simulink library "three_phase_bridge_three_level_ttype_ideal_switch"  (R2026a)
settings: Solver=VariableStepAuto
libraries: fl_lib x60, nesl_utility x36
settings Model: Creator=pwr-control  LastModifiedBy=pwr-control

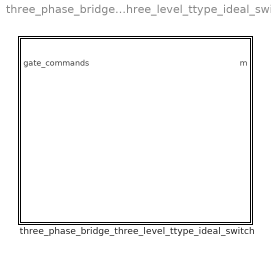
== system three_phase_bridge_three_level_ttype_ideal_switch ==
  three_phase_bridge_three_level_ttype_ideal_switch : Subsystem  mask(three_phase_bridge_three_level_ttype_ideal_switch){Rds_on=1.85e-3, Vdon_diode=0.35, Rdon_diode=1.85e-3, Csnubber=6e-9, Rsnubber=3e3, Vth=7.5}
      mask prompts: Rds_on "On-state resistance of the switch [Ohm]"; Vdon_diode "Diode forward voltage [V]"; Rdon_diode "Diode on-state resistance [Ohm]"; Csnubber "RC snubber capacitance [F]"; Rsnubber "RC snubber resistance [Ohm]"; Vth "Gate threshold: the switch is closed when the gate command is above Vth"
      mask help: Three-phase bridge, three-level T-type, ideal switch devices. Ideal switch cells: Simscape Foundation controlled switch (closed when the gate command is above Vth) with antiparallel piecewise-linear diode and RC snubber. No losses are computed; the cell measures the device current (positive from collector/drain to emitter/source, diode current negative) and the device voltage. Bus m: switch_current_Qk, switch_voltage_Qk. Ports: gate_commands (bus from the three-level PWM modulators of masked_models/modulators), m (measurement bus), left dc terminals udc(+) / np / udc(-), right ac terminals u / v / w. Device numbering: see three_phase_bridge/README.md.
      mask Help: web('https://github.com/pwr-control/library/blob/dev/library/masked_models/semiconductors_bridges/three_phase_bridge/README.md', '-browser')
      mask DialogControl ParameterGroupVar Prompt: Switch and diode
      mask DialogControl ParameterGroupVar1 Prompt: RC snubber
      mask Display:
      | disp(sprintf('three-phase bridge\nT-type 3 levels\nideal switch'))
      | port_label('input', 1, 'gate_commands')
      | port_label('output', 1, 'm')
      | port_label('LConn', 1, 'udc(+)')
      | port_label('LConn', 2, 'np')
      | port_label('LConn', 3, 'udc(-)')
      | port_label('RConn', 1, 'u')
      | port_label('RConn', 2, 'v')
      | port_label('RConn', 3, 'w')

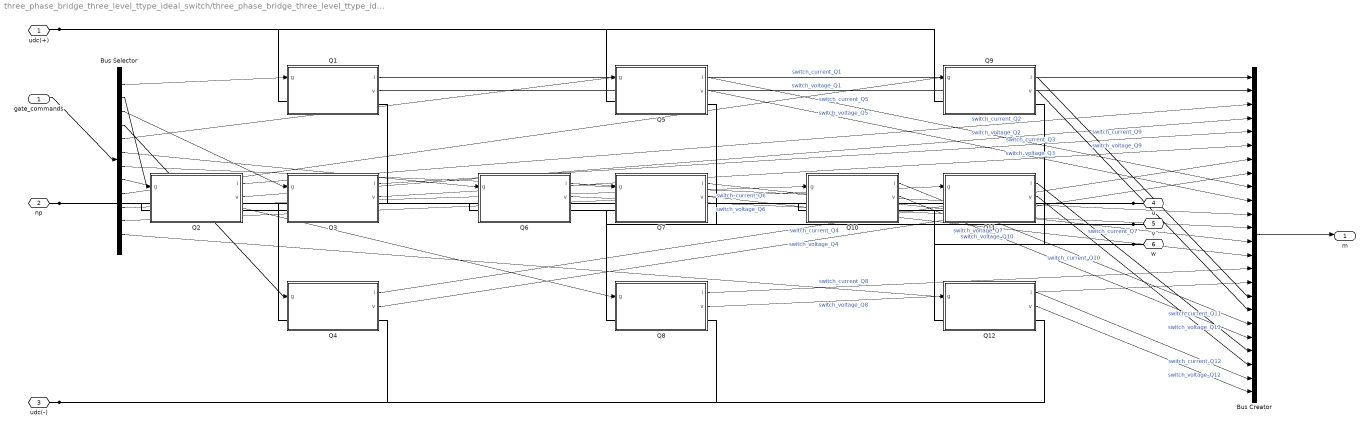
== system three_phase_bridge_three_level_ttype_ideal_switch/three_phase_bridge_three_level_ttype_ideal_switch ==
  gate_commands : Inport
  Bus Selector : BusSelector  OutputSignals=gate_cmds_phu.cmd_gate_Q1,gate_cmds_phu.cmd_gate_Q2,gate_cmds_phu.cmd_gate_Q3,gate_cmds_phu.cmd_gate_Q4,gate_cmds_phv.cmd_gate_Q1,gate_cmds_phv.cmd_gate_Q2,gate_cmds_phv.cmd_gate_Q3,gate_cmds_phv.cmd_gate_Q4,gate_cmds_phw.cmd_gate_Q1,gate_cmds_phw.cmd_gate_Q2,gate_cmds_phw.cmd_gate_Q3,gate_cmds_phw.cmd_gate_Q4
  udc(+) : PMIOPort  Side=Left
  np : PMIOPort  Port=2  Side=Left
  udc(-) : PMIOPort  Port=3  Side=Left
  u : PMIOPort  Port=4  Side=Right
  v : PMIOPort  Port=5  Side=Right
  w : PMIOPort  Port=6  Side=Right
  Bus Creator : BusCreator  Inputs=24
  m : Outport
  Q1 : Subsystem
  Q2 : Subsystem
  Q3 : Subsystem
  Q4 : Subsystem
  Q5 : Subsystem
  Q6 : Subsystem
  Q7 : Subsystem
  Q8 : Subsystem
  Q9 : Subsystem
  Q10 : Subsystem
  Q11 : Subsystem
  Q12 : Subsystem
  wires:
  gate_commands/1 -> Bus Selector/1
  Bus Creator/1 -> m/1
  Bus Selector/1 -> Q1/1(g)
  Q1/1(i) -> Bus Creator/1  "switch_current_Q1"
  Q1/2(v) -> Bus Creator/2  "switch_voltage_Q1"
  Bus Selector/2 -> Q2/1(g)
  Q2/1(i) -> Bus Creator/3  "switch_current_Q2"
  Q2/2(v) -> Bus Creator/4  "switch_voltage_Q2"
  Bus Selector/3 -> Q3/1(g)
  Q3/1(i) -> Bus Creator/5  "switch_current_Q3"
  Q3/2(v) -> Bus Creator/6  "switch_voltage_Q3"
  Bus Selector/4 -> Q4/1(g)
  Q4/1(i) -> Bus Creator/7  "switch_current_Q4"
  Q4/2(v) -> Bus Creator/8  "switch_voltage_Q4"
  Bus Selector/5 -> Q5/1(g)
  Q5/1(i) -> Bus Creator/9  "switch_current_Q5"
  Q5/2(v) -> Bus Creator/10  "switch_voltage_Q5"
  Bus Selector/6 -> Q6/1(g)
  Q6/1(i) -> Bus Creator/11  "switch_current_Q6"
  Q6/2(v) -> Bus Creator/12  "switch_voltage_Q6"
  Bus Selector/7 -> Q7/1(g)
  Q7/1(i) -> Bus Creator/13  "switch_current_Q7"
  Q7/2(v) -> Bus Creator/14  "switch_voltage_Q7"
  Bus Selector/8 -> Q8/1(g)
  Q8/1(i) -> Bus Creator/15  "switch_current_Q8"
  Q8/2(v) -> Bus Creator/16  "switch_voltage_Q8"
  Bus Selector/9 -> Q9/1(g)
  Q9/1(i) -> Bus Creator/17  "switch_current_Q9"
  Q9/2(v) -> Bus Creator/18  "switch_voltage_Q9"
  Bus Selector/10 -> Q10/1(g)
  Q10/1(i) -> Bus Creator/19  "switch_current_Q10"
  Q10/2(v) -> Bus Creator/20  "switch_voltage_Q10"
  Bus Selector/11 -> Q11/1(g)
  Q11/1(i) -> Bus Creator/21  "switch_current_Q11"
  Q11/2(v) -> Bus Creator/22  "switch_voltage_Q11"
  Bus Selector/12 -> Q12/1(g)
  Q12/1(i) -> Bus Creator/23  "switch_current_Q12"
  Q12/2(v) -> Bus Creator/24  "switch_voltage_Q12"
  connections:
  Q2/RConn1 -- Q3/RConn1
  u/RConn1 -- Q1/RConn1 -- Q4/LConn1 -- Q3/LConn1
  Q6/RConn1 -- Q7/RConn1
  v/RConn1 -- Q5/RConn1 -- Q8/LConn1 -- Q7/LConn1
  Q10/RConn1 -- Q11/RConn1
  w/RConn1 -- Q9/RConn1 -- Q12/LConn1 -- Q11/LConn1
  udc(+)/RConn1 -- Q1/LConn1 -- Q5/LConn1 -- Q9/LConn1
  udc(-)/RConn1 -- Q4/RConn1 -- Q8/RConn1 -- Q12/RConn1
  np/RConn1 -- Q2/LConn1 -- Q6/LConn1 -- Q10/LConn1

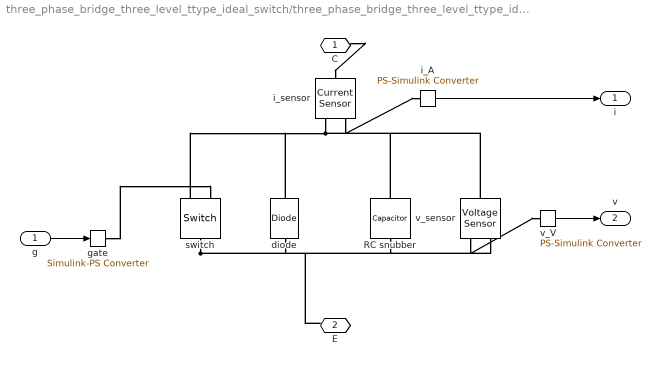
== system three_phase_bridge_three_level_ttype_ideal_switch/three_phase_bridge_three_level_ttype_ideal_switch/Q1 ==
  g : Inport
  gate : nesl_utility/Simulink-PS Converter  PhysicalDomain=network_engine_domain  SubClassName=ps_input  LeftPortType=input  RightPortType=output  PseudoPeriodic=off  Frequencies=[]  NoiseDistribution=none  NoiseParameters=[]  Unit=1  AffineConversion=off  FilteringAndDerivatives=provide  SimscapeFilterOrder=1  InputFilterTimeConstant=0.001  UdotUserProvided=0
  C : PMIOPort  Side=Left
  i_sensor : fl_lib/Electrical/Electrical Sensors/Current Sensor
  switch : fl_lib/Electrical/Electrical Elements/Switch  R_closed=Rds_on Ohm  G_open=1e-8 1/Ohm  Threshold=Vth  i_specify=off  i_priority=None  i=0 A  i_nominal_specify=off  i_nominal_value=1  i_nominal_unit=A  v_specify=off  v_priority=None  v=0 V  v_nominal_specify=off  v_nominal_value=1  v_nominal_unit=V
  diode : fl_lib/Electrical/Electrical Elements/Diode  Vf=Vdon_diode V  Ron=Rdon_diode Ohm  Goff=1e-8 1/Ohm  i_specify=off  i_priority=None  i=0 A  i_nominal_specify=off  i_nominal_value=1  i_nominal_unit=A  v_specify=off  v_priority=None  v=0 V  v_nominal_specify=off  v_nominal_value=1  v_nominal_unit=V
  RC snubber : fl_lib/Electrical/Electrical Elements/Capacitor  c=Csnubber F  r=Rsnubber Ohm  g=0 1/Ohm  i_specify=off  i_priority=None  i=0 A  i_nominal_specify=off  i_nominal_value=1  i_nominal_unit=A  v_specify=off  v_priority=None  v=0 V  v_nominal_specify=off  v_nominal_value=1  v_nominal_unit=V  vc_specify=off  vc_priority=High  vc=0 V  vc_nominal_specify=off  vc_nominal_value=1  vc_nominal_unit=V
  v_sensor : fl_lib/Electrical/Electrical Sensors/Voltage Sensor
  E : PMIOPort  Port=2  Side=Right
  i_A : nesl_utility/PS-Simulink Converter  PhysicalDomain=network_engine_domain  SubClassName=ps_output  LeftPortType=input  RightPortType=output  PseudoPeriodic=off  Frequencies=[]  VectorFormat=1-D array  Unit=A  AffineConversion=off
  v_V : nesl_utility/PS-Simulink Converter  PhysicalDomain=network_engine_domain  SubClassName=ps_output  LeftPortType=input  RightPortType=output  PseudoPeriodic=off  Frequencies=[]  VectorFormat=1-D array  Unit=V  AffineConversion=off
  i : Outport
  v : Outport  Port=2
  wires:
  g/1 -> gate/1
  i_A/1 -> i/1
  v_V/1 -> v/1
  connections:
  gate/RConn1 -- switch/RConn1
  C/RConn1 -- i_sensor/LConn1
  i_sensor/RConn2 -- switch/RConn2 -- diode/RConn1 -- RC snubber/LConn1 -- v_sensor/LConn1
  switch/LConn1 -- diode/LConn1 -- RC snubber/RConn1 -- v_sensor/RConn2 -- E/RConn1
  i_sensor/RConn1 -- i_A/LConn1
  v_sensor/RConn1 -- v_V/LConn1

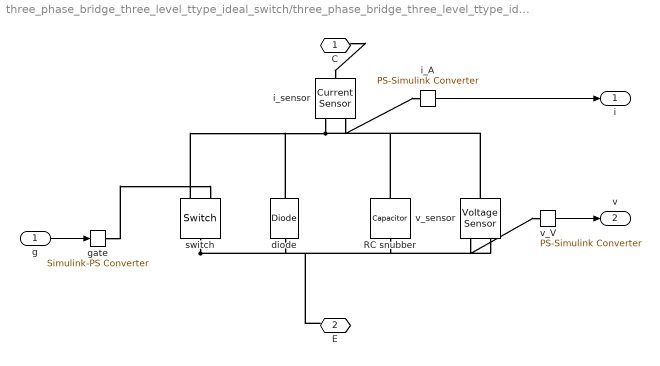
== system three_phase_bridge_three_level_ttype_ideal_switch/three_phase_bridge_three_level_ttype_ideal_switch/Q2 ==
  g : Inport
  gate : nesl_utility/Simulink-PS Converter  PhysicalDomain=network_engine_domain  SubClassName=ps_input  LeftPortType=input  RightPortType=output  PseudoPeriodic=off  Frequencies=[]  NoiseDistribution=none  NoiseParameters=[]  Unit=1  AffineConversion=off  FilteringAndDerivatives=provide  SimscapeFilterOrder=1  InputFilterTimeConstant=0.001  UdotUserProvided=0
  C : PMIOPort  Side=Left
  i_sensor : fl_lib/Electrical/Electrical Sensors/Current Sensor
  switch : fl_lib/Electrical/Electrical Elements/Switch  R_closed=Rds_on Ohm  G_open=1e-8 1/Ohm  Threshold=Vth  i_specify=off  i_priority=None  i=0 A  i_nominal_specify=off  i_nominal_value=1  i_nominal_unit=A  v_specify=off  v_priority=None  v=0 V  v_nominal_specify=off  v_nominal_value=1  v_nominal_unit=V
  diode : fl_lib/Electrical/Electrical Elements/Diode  Vf=Vdon_diode V  Ron=Rdon_diode Ohm  Goff=1e-8 1/Ohm  i_specify=off  i_priority=None  i=0 A  i_nominal_specify=off  i_nominal_value=1  i_nominal_unit=A  v_specify=off  v_priority=None  v=0 V  v_nominal_specify=off  v_nominal_value=1  v_nominal_unit=V
  RC snubber : fl_lib/Electrical/Electrical Elements/Capacitor  c=Csnubber F  r=Rsnubber Ohm  g=0 1/Ohm  i_specify=off  i_priority=None  i=0 A  i_nominal_specify=off  i_nominal_value=1  i_nominal_unit=A  v_specify=off  v_priority=None  v=0 V  v_nominal_specify=off  v_nominal_value=1  v_nominal_unit=V  vc_specify=off  vc_priority=High  vc=0 V  vc_nominal_specify=off  vc_nominal_value=1  vc_nominal_unit=V
  v_sensor : fl_lib/Electrical/Electrical Sensors/Voltage Sensor
  E : PMIOPort  Port=2  Side=Right
  i_A : nesl_utility/PS-Simulink Converter  PhysicalDomain=network_engine_domain  SubClassName=ps_output  LeftPortType=input  RightPortType=output  PseudoPeriodic=off  Frequencies=[]  VectorFormat=1-D array  Unit=A  AffineConversion=off
  v_V : nesl_utility/PS-Simulink Converter  PhysicalDomain=network_engine_domain  SubClassName=ps_output  LeftPortType=input  RightPortType=output  PseudoPeriodic=off  Frequencies=[]  VectorFormat=1-D array  Unit=V  AffineConversion=off
  i : Outport
  v : Outport  Port=2
  wires:
  g/1 -> gate/1
  i_A/1 -> i/1
  v_V/1 -> v/1
  connections:
  gate/RConn1 -- switch/RConn1
  C/RConn1 -- i_sensor/LConn1
  i_sensor/RConn2 -- switch/RConn2 -- diode/RConn1 -- RC snubber/LConn1 -- v_sensor/LConn1
  switch/LConn1 -- diode/LConn1 -- RC snubber/RConn1 -- v_sensor/RConn2 -- E/RConn1
  i_sensor/RConn1 -- i_A/LConn1
  v_sensor/RConn1 -- v_V/LConn1

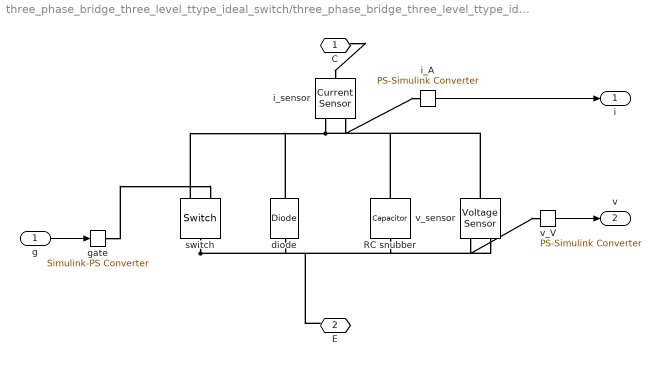
== system three_phase_bridge_three_level_ttype_ideal_switch/three_phase_bridge_three_level_ttype_ideal_switch/Q3 ==
  g : Inport
  gate : nesl_utility/Simulink-PS Converter  PhysicalDomain=network_engine_domain  SubClassName=ps_input  LeftPortType=input  RightPortType=output  PseudoPeriodic=off  Frequencies=[]  NoiseDistribution=none  NoiseParameters=[]  Unit=1  AffineConversion=off  FilteringAndDerivatives=provide  SimscapeFilterOrder=1  InputFilterTimeConstant=0.001  UdotUserProvided=0
  C : PMIOPort  Side=Left
  i_sensor : fl_lib/Electrical/Electrical Sensors/Current Sensor
  switch : fl_lib/Electrical/Electrical Elements/Switch  R_closed=Rds_on Ohm  G_open=1e-8 1/Ohm  Threshold=Vth  i_specify=off  i_priority=None  i=0 A  i_nominal_specify=off  i_nominal_value=1  i_nominal_unit=A  v_specify=off  v_priority=None  v=0 V  v_nominal_specify=off  v_nominal_value=1  v_nominal_unit=V
  diode : fl_lib/Electrical/Electrical Elements/Diode  Vf=Vdon_diode V  Ron=Rdon_diode Ohm  Goff=1e-8 1/Ohm  i_specify=off  i_priority=None  i=0 A  i_nominal_specify=off  i_nominal_value=1  i_nominal_unit=A  v_specify=off  v_priority=None  v=0 V  v_nominal_specify=off  v_nominal_value=1  v_nominal_unit=V
  RC snubber : fl_lib/Electrical/Electrical Elements/Capacitor  c=Csnubber F  r=Rsnubber Ohm  g=0 1/Ohm  i_specify=off  i_priority=None  i=0 A  i_nominal_specify=off  i_nominal_value=1  i_nominal_unit=A  v_specify=off  v_priority=None  v=0 V  v_nominal_specify=off  v_nominal_value=1  v_nominal_unit=V  vc_specify=off  vc_priority=High  vc=0 V  vc_nominal_specify=off  vc_nominal_value=1  vc_nominal_unit=V
  v_sensor : fl_lib/Electrical/Electrical Sensors/Voltage Sensor
  E : PMIOPort  Port=2  Side=Right
  i_A : nesl_utility/PS-Simulink Converter  PhysicalDomain=network_engine_domain  SubClassName=ps_output  LeftPortType=input  RightPortType=output  PseudoPeriodic=off  Frequencies=[]  VectorFormat=1-D array  Unit=A  AffineConversion=off
  v_V : nesl_utility/PS-Simulink Converter  PhysicalDomain=network_engine_domain  SubClassName=ps_output  LeftPortType=input  RightPortType=output  PseudoPeriodic=off  Frequencies=[]  VectorFormat=1-D array  Unit=V  AffineConversion=off
  i : Outport
  v : Outport  Port=2
  wires:
  g/1 -> gate/1
  i_A/1 -> i/1
  v_V/1 -> v/1
  connections:
  gate/RConn1 -- switch/RConn1
  C/RConn1 -- i_sensor/LConn1
  i_sensor/RConn2 -- switch/RConn2 -- diode/RConn1 -- RC snubber/LConn1 -- v_sensor/LConn1
  switch/LConn1 -- diode/LConn1 -- RC snubber/RConn1 -- v_sensor/RConn2 -- E/RConn1
  i_sensor/RConn1 -- i_A/LConn1
  v_sensor/RConn1 -- v_V/LConn1

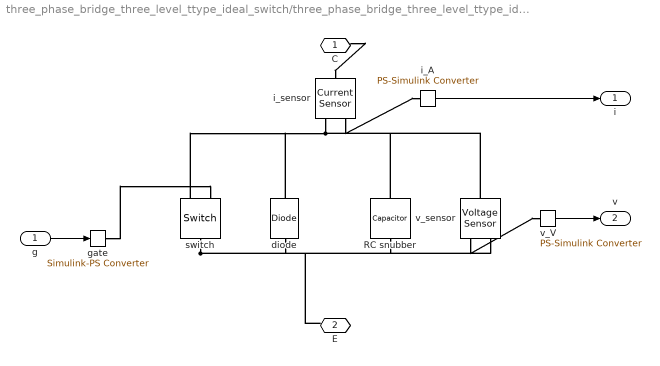
== system three_phase_bridge_three_level_ttype_ideal_switch/three_phase_bridge_three_level_ttype_ideal_switch/Q4 ==
  g : Inport
  gate : nesl_utility/Simulink-PS Converter  PhysicalDomain=network_engine_domain  SubClassName=ps_input  LeftPortType=input  RightPortType=output  PseudoPeriodic=off  Frequencies=[]  NoiseDistribution=none  NoiseParameters=[]  Unit=1  AffineConversion=off  FilteringAndDerivatives=provide  SimscapeFilterOrder=1  InputFilterTimeConstant=0.001  UdotUserProvided=0
  C : PMIOPort  Side=Left
  i_sensor : fl_lib/Electrical/Electrical Sensors/Current Sensor
  switch : fl_lib/Electrical/Electrical Elements/Switch  R_closed=Rds_on Ohm  G_open=1e-8 1/Ohm  Threshold=Vth  i_specify=off  i_priority=None  i=0 A  i_nominal_specify=off  i_nominal_value=1  i_nominal_unit=A  v_specify=off  v_priority=None  v=0 V  v_nominal_specify=off  v_nominal_value=1  v_nominal_unit=V
  diode : fl_lib/Electrical/Electrical Elements/Diode  Vf=Vdon_diode V  Ron=Rdon_diode Ohm  Goff=1e-8 1/Ohm  i_specify=off  i_priority=None  i=0 A  i_nominal_specify=off  i_nominal_value=1  i_nominal_unit=A  v_specify=off  v_priority=None  v=0 V  v_nominal_specify=off  v_nominal_value=1  v_nominal_unit=V
  RC snubber : fl_lib/Electrical/Electrical Elements/Capacitor  c=Csnubber F  r=Rsnubber Ohm  g=0 1/Ohm  i_specify=off  i_priority=None  i=0 A  i_nominal_specify=off  i_nominal_value=1  i_nominal_unit=A  v_specify=off  v_priority=None  v=0 V  v_nominal_specify=off  v_nominal_value=1  v_nominal_unit=V  vc_specify=off  vc_priority=High  vc=0 V  vc_nominal_specify=off  vc_nominal_value=1  vc_nominal_unit=V
  v_sensor : fl_lib/Electrical/Electrical Sensors/Voltage Sensor
  E : PMIOPort  Port=2  Side=Right
  i_A : nesl_utility/PS-Simulink Converter  PhysicalDomain=network_engine_domain  SubClassName=ps_output  LeftPortType=input  RightPortType=output  PseudoPeriodic=off  Frequencies=[]  VectorFormat=1-D array  Unit=A  AffineConversion=off
  v_V : nesl_utility/PS-Simulink Converter  PhysicalDomain=network_engine_domain  SubClassName=ps_output  LeftPortType=input  RightPortType=output  PseudoPeriodic=off  Frequencies=[]  VectorFormat=1-D array  Unit=V  AffineConversion=off
  i : Outport
  v : Outport  Port=2
  wires:
  g/1 -> gate/1
  i_A/1 -> i/1
  v_V/1 -> v/1
  connections:
  gate/RConn1 -- switch/RConn1
  C/RConn1 -- i_sensor/LConn1
  i_sensor/RConn2 -- switch/RConn2 -- diode/RConn1 -- RC snubber/LConn1 -- v_sensor/LConn1
  switch/LConn1 -- diode/LConn1 -- RC snubber/RConn1 -- v_sensor/RConn2 -- E/RConn1
  i_sensor/RConn1 -- i_A/LConn1
  v_sensor/RConn1 -- v_V/LConn1

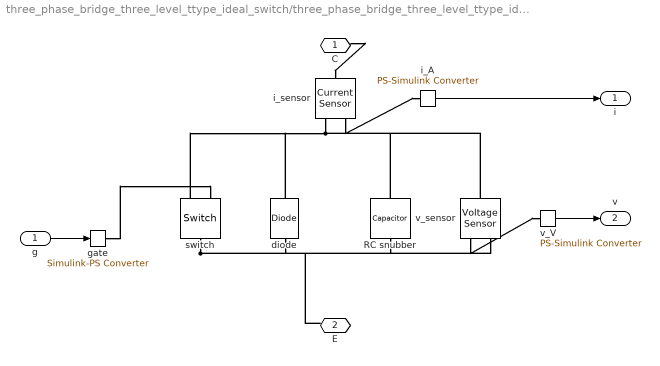
== system three_phase_bridge_three_level_ttype_ideal_switch/three_phase_bridge_three_level_ttype_ideal_switch/Q5 ==
  g : Inport
  gate : nesl_utility/Simulink-PS Converter  PhysicalDomain=network_engine_domain  SubClassName=ps_input  LeftPortType=input  RightPortType=output  PseudoPeriodic=off  Frequencies=[]  NoiseDistribution=none  NoiseParameters=[]  Unit=1  AffineConversion=off  FilteringAndDerivatives=provide  SimscapeFilterOrder=1  InputFilterTimeConstant=0.001  UdotUserProvided=0
  C : PMIOPort  Side=Left
  i_sensor : fl_lib/Electrical/Electrical Sensors/Current Sensor
  switch : fl_lib/Electrical/Electrical Elements/Switch  R_closed=Rds_on Ohm  G_open=1e-8 1/Ohm  Threshold=Vth  i_specify=off  i_priority=None  i=0 A  i_nominal_specify=off  i_nominal_value=1  i_nominal_unit=A  v_specify=off  v_priority=None  v=0 V  v_nominal_specify=off  v_nominal_value=1  v_nominal_unit=V
  diode : fl_lib/Electrical/Electrical Elements/Diode  Vf=Vdon_diode V  Ron=Rdon_diode Ohm  Goff=1e-8 1/Ohm  i_specify=off  i_priority=None  i=0 A  i_nominal_specify=off  i_nominal_value=1  i_nominal_unit=A  v_specify=off  v_priority=None  v=0 V  v_nominal_specify=off  v_nominal_value=1  v_nominal_unit=V
  RC snubber : fl_lib/Electrical/Electrical Elements/Capacitor  c=Csnubber F  r=Rsnubber Ohm  g=0 1/Ohm  i_specify=off  i_priority=None  i=0 A  i_nominal_specify=off  i_nominal_value=1  i_nominal_unit=A  v_specify=off  v_priority=None  v=0 V  v_nominal_specify=off  v_nominal_value=1  v_nominal_unit=V  vc_specify=off  vc_priority=High  vc=0 V  vc_nominal_specify=off  vc_nominal_value=1  vc_nominal_unit=V
  v_sensor : fl_lib/Electrical/Electrical Sensors/Voltage Sensor
  E : PMIOPort  Port=2  Side=Right
  i_A : nesl_utility/PS-Simulink Converter  PhysicalDomain=network_engine_domain  SubClassName=ps_output  LeftPortType=input  RightPortType=output  PseudoPeriodic=off  Frequencies=[]  VectorFormat=1-D array  Unit=A  AffineConversion=off
  v_V : nesl_utility/PS-Simulink Converter  PhysicalDomain=network_engine_domain  SubClassName=ps_output  LeftPortType=input  RightPortType=output  PseudoPeriodic=off  Frequencies=[]  VectorFormat=1-D array  Unit=V  AffineConversion=off
  i : Outport
  v : Outport  Port=2
  wires:
  g/1 -> gate/1
  i_A/1 -> i/1
  v_V/1 -> v/1
  connections:
  gate/RConn1 -- switch/RConn1
  C/RConn1 -- i_sensor/LConn1
  i_sensor/RConn2 -- switch/RConn2 -- diode/RConn1 -- RC snubber/LConn1 -- v_sensor/LConn1
  switch/LConn1 -- diode/LConn1 -- RC snubber/RConn1 -- v_sensor/RConn2 -- E/RConn1
  i_sensor/RConn1 -- i_A/LConn1
  v_sensor/RConn1 -- v_V/LConn1

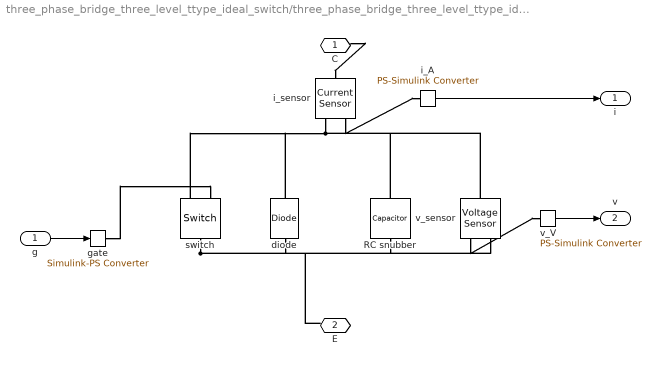
== system three_phase_bridge_three_level_ttype_ideal_switch/three_phase_bridge_three_level_ttype_ideal_switch/Q6 ==
  g : Inport
  gate : nesl_utility/Simulink-PS Converter  PhysicalDomain=network_engine_domain  SubClassName=ps_input  LeftPortType=input  RightPortType=output  PseudoPeriodic=off  Frequencies=[]  NoiseDistribution=none  NoiseParameters=[]  Unit=1  AffineConversion=off  FilteringAndDerivatives=provide  SimscapeFilterOrder=1  InputFilterTimeConstant=0.001  UdotUserProvided=0
  C : PMIOPort  Side=Left
  i_sensor : fl_lib/Electrical/Electrical Sensors/Current Sensor
  switch : fl_lib/Electrical/Electrical Elements/Switch  R_closed=Rds_on Ohm  G_open=1e-8 1/Ohm  Threshold=Vth  i_specify=off  i_priority=None  i=0 A  i_nominal_specify=off  i_nominal_value=1  i_nominal_unit=A  v_specify=off  v_priority=None  v=0 V  v_nominal_specify=off  v_nominal_value=1  v_nominal_unit=V
  diode : fl_lib/Electrical/Electrical Elements/Diode  Vf=Vdon_diode V  Ron=Rdon_diode Ohm  Goff=1e-8 1/Ohm  i_specify=off  i_priority=None  i=0 A  i_nominal_specify=off  i_nominal_value=1  i_nominal_unit=A  v_specify=off  v_priority=None  v=0 V  v_nominal_specify=off  v_nominal_value=1  v_nominal_unit=V
  RC snubber : fl_lib/Electrical/Electrical Elements/Capacitor  c=Csnubber F  r=Rsnubber Ohm  g=0 1/Ohm  i_specify=off  i_priority=None  i=0 A  i_nominal_specify=off  i_nominal_value=1  i_nominal_unit=A  v_specify=off  v_priority=None  v=0 V  v_nominal_specify=off  v_nominal_value=1  v_nominal_unit=V  vc_specify=off  vc_priority=High  vc=0 V  vc_nominal_specify=off  vc_nominal_value=1  vc_nominal_unit=V
  v_sensor : fl_lib/Electrical/Electrical Sensors/Voltage Sensor
  E : PMIOPort  Port=2  Side=Right
  i_A : nesl_utility/PS-Simulink Converter  PhysicalDomain=network_engine_domain  SubClassName=ps_output  LeftPortType=input  RightPortType=output  PseudoPeriodic=off  Frequencies=[]  VectorFormat=1-D array  Unit=A  AffineConversion=off
  v_V : nesl_utility/PS-Simulink Converter  PhysicalDomain=network_engine_domain  SubClassName=ps_output  LeftPortType=input  RightPortType=output  PseudoPeriodic=off  Frequencies=[]  VectorFormat=1-D array  Unit=V  AffineConversion=off
  i : Outport
  v : Outport  Port=2
  wires:
  g/1 -> gate/1
  i_A/1 -> i/1
  v_V/1 -> v/1
  connections:
  gate/RConn1 -- switch/RConn1
  C/RConn1 -- i_sensor/LConn1
  i_sensor/RConn2 -- switch/RConn2 -- diode/RConn1 -- RC snubber/LConn1 -- v_sensor/LConn1
  switch/LConn1 -- diode/LConn1 -- RC snubber/RConn1 -- v_sensor/RConn2 -- E/RConn1
  i_sensor/RConn1 -- i_A/LConn1
  v_sensor/RConn1 -- v_V/LConn1

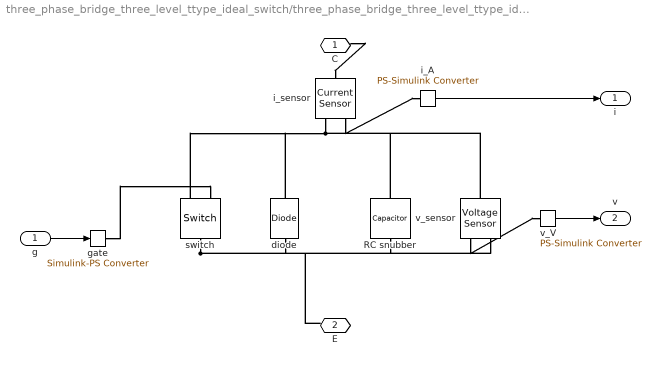
== system three_phase_bridge_three_level_ttype_ideal_switch/three_phase_bridge_three_level_ttype_ideal_switch/Q7 ==
  g : Inport
  gate : nesl_utility/Simulink-PS Converter  PhysicalDomain=network_engine_domain  SubClassName=ps_input  LeftPortType=input  RightPortType=output  PseudoPeriodic=off  Frequencies=[]  NoiseDistribution=none  NoiseParameters=[]  Unit=1  AffineConversion=off  FilteringAndDerivatives=provide  SimscapeFilterOrder=1  InputFilterTimeConstant=0.001  UdotUserProvided=0
  C : PMIOPort  Side=Left
  i_sensor : fl_lib/Electrical/Electrical Sensors/Current Sensor
  switch : fl_lib/Electrical/Electrical Elements/Switch  R_closed=Rds_on Ohm  G_open=1e-8 1/Ohm  Threshold=Vth  i_specify=off  i_priority=None  i=0 A  i_nominal_specify=off  i_nominal_value=1  i_nominal_unit=A  v_specify=off  v_priority=None  v=0 V  v_nominal_specify=off  v_nominal_value=1  v_nominal_unit=V
  diode : fl_lib/Electrical/Electrical Elements/Diode  Vf=Vdon_diode V  Ron=Rdon_diode Ohm  Goff=1e-8 1/Ohm  i_specify=off  i_priority=None  i=0 A  i_nominal_specify=off  i_nominal_value=1  i_nominal_unit=A  v_specify=off  v_priority=None  v=0 V  v_nominal_specify=off  v_nominal_value=1  v_nominal_unit=V
  RC snubber : fl_lib/Electrical/Electrical Elements/Capacitor  c=Csnubber F  r=Rsnubber Ohm  g=0 1/Ohm  i_specify=off  i_priority=None  i=0 A  i_nominal_specify=off  i_nominal_value=1  i_nominal_unit=A  v_specify=off  v_priority=None  v=0 V  v_nominal_specify=off  v_nominal_value=1  v_nominal_unit=V  vc_specify=off  vc_priority=High  vc=0 V  vc_nominal_specify=off  vc_nominal_value=1  vc_nominal_unit=V
  v_sensor : fl_lib/Electrical/Electrical Sensors/Voltage Sensor
  E : PMIOPort  Port=2  Side=Right
  i_A : nesl_utility/PS-Simulink Converter  PhysicalDomain=network_engine_domain  SubClassName=ps_output  LeftPortType=input  RightPortType=output  PseudoPeriodic=off  Frequencies=[]  VectorFormat=1-D array  Unit=A  AffineConversion=off
  v_V : nesl_utility/PS-Simulink Converter  PhysicalDomain=network_engine_domain  SubClassName=ps_output  LeftPortType=input  RightPortType=output  PseudoPeriodic=off  Frequencies=[]  VectorFormat=1-D array  Unit=V  AffineConversion=off
  i : Outport
  v : Outport  Port=2
  wires:
  g/1 -> gate/1
  i_A/1 -> i/1
  v_V/1 -> v/1
  connections:
  gate/RConn1 -- switch/RConn1
  C/RConn1 -- i_sensor/LConn1
  i_sensor/RConn2 -- switch/RConn2 -- diode/RConn1 -- RC snubber/LConn1 -- v_sensor/LConn1
  switch/LConn1 -- diode/LConn1 -- RC snubber/RConn1 -- v_sensor/RConn2 -- E/RConn1
  i_sensor/RConn1 -- i_A/LConn1
  v_sensor/RConn1 -- v_V/LConn1

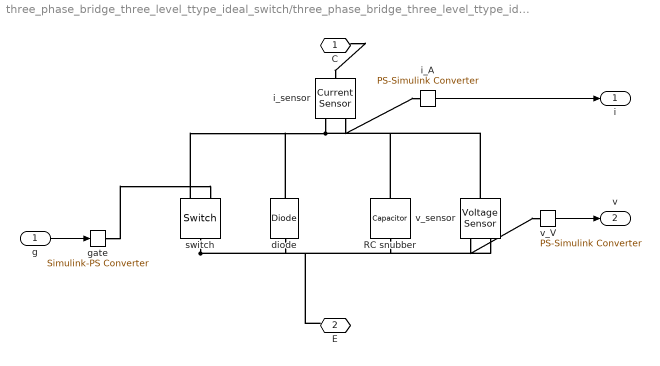
== system three_phase_bridge_three_level_ttype_ideal_switch/three_phase_bridge_three_level_ttype_ideal_switch/Q8 ==
  g : Inport
  gate : nesl_utility/Simulink-PS Converter  PhysicalDomain=network_engine_domain  SubClassName=ps_input  LeftPortType=input  RightPortType=output  PseudoPeriodic=off  Frequencies=[]  NoiseDistribution=none  NoiseParameters=[]  Unit=1  AffineConversion=off  FilteringAndDerivatives=provide  SimscapeFilterOrder=1  InputFilterTimeConstant=0.001  UdotUserProvided=0
  C : PMIOPort  Side=Left
  i_sensor : fl_lib/Electrical/Electrical Sensors/Current Sensor
  switch : fl_lib/Electrical/Electrical Elements/Switch  R_closed=Rds_on Ohm  G_open=1e-8 1/Ohm  Threshold=Vth  i_specify=off  i_priority=None  i=0 A  i_nominal_specify=off  i_nominal_value=1  i_nominal_unit=A  v_specify=off  v_priority=None  v=0 V  v_nominal_specify=off  v_nominal_value=1  v_nominal_unit=V
  diode : fl_lib/Electrical/Electrical Elements/Diode  Vf=Vdon_diode V  Ron=Rdon_diode Ohm  Goff=1e-8 1/Ohm  i_specify=off  i_priority=None  i=0 A  i_nominal_specify=off  i_nominal_value=1  i_nominal_unit=A  v_specify=off  v_priority=None  v=0 V  v_nominal_specify=off  v_nominal_value=1  v_nominal_unit=V
  RC snubber : fl_lib/Electrical/Electrical Elements/Capacitor  c=Csnubber F  r=Rsnubber Ohm  g=0 1/Ohm  i_specify=off  i_priority=None  i=0 A  i_nominal_specify=off  i_nominal_value=1  i_nominal_unit=A  v_specify=off  v_priority=None  v=0 V  v_nominal_specify=off  v_nominal_value=1  v_nominal_unit=V  vc_specify=off  vc_priority=High  vc=0 V  vc_nominal_specify=off  vc_nominal_value=1  vc_nominal_unit=V
  v_sensor : fl_lib/Electrical/Electrical Sensors/Voltage Sensor
  E : PMIOPort  Port=2  Side=Right
  i_A : nesl_utility/PS-Simulink Converter  PhysicalDomain=network_engine_domain  SubClassName=ps_output  LeftPortType=input  RightPortType=output  PseudoPeriodic=off  Frequencies=[]  VectorFormat=1-D array  Unit=A  AffineConversion=off
  v_V : nesl_utility/PS-Simulink Converter  PhysicalDomain=network_engine_domain  SubClassName=ps_output  LeftPortType=input  RightPortType=output  PseudoPeriodic=off  Frequencies=[]  VectorFormat=1-D array  Unit=V  AffineConversion=off
  i : Outport
  v : Outport  Port=2
  wires:
  g/1 -> gate/1
  i_A/1 -> i/1
  v_V/1 -> v/1
  connections:
  gate/RConn1 -- switch/RConn1
  C/RConn1 -- i_sensor/LConn1
  i_sensor/RConn2 -- switch/RConn2 -- diode/RConn1 -- RC snubber/LConn1 -- v_sensor/LConn1
  switch/LConn1 -- diode/LConn1 -- RC snubber/RConn1 -- v_sensor/RConn2 -- E/RConn1
  i_sensor/RConn1 -- i_A/LConn1
  v_sensor/RConn1 -- v_V/LConn1

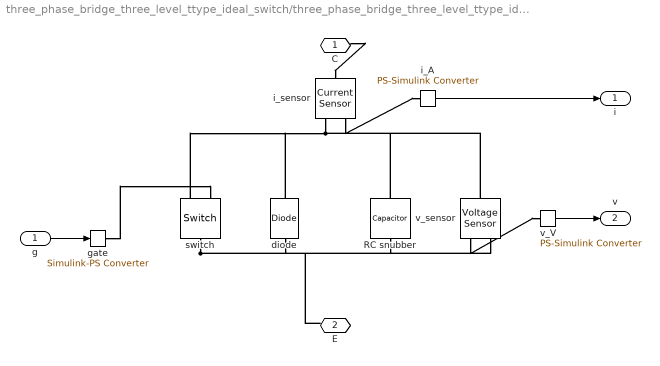
== system three_phase_bridge_three_level_ttype_ideal_switch/three_phase_bridge_three_level_ttype_ideal_switch/Q9 ==
  g : Inport
  gate : nesl_utility/Simulink-PS Converter  PhysicalDomain=network_engine_domain  SubClassName=ps_input  LeftPortType=input  RightPortType=output  PseudoPeriodic=off  Frequencies=[]  NoiseDistribution=none  NoiseParameters=[]  Unit=1  AffineConversion=off  FilteringAndDerivatives=provide  SimscapeFilterOrder=1  InputFilterTimeConstant=0.001  UdotUserProvided=0
  C : PMIOPort  Side=Left
  i_sensor : fl_lib/Electrical/Electrical Sensors/Current Sensor
  switch : fl_lib/Electrical/Electrical Elements/Switch  R_closed=Rds_on Ohm  G_open=1e-8 1/Ohm  Threshold=Vth  i_specify=off  i_priority=None  i=0 A  i_nominal_specify=off  i_nominal_value=1  i_nominal_unit=A  v_specify=off  v_priority=None  v=0 V  v_nominal_specify=off  v_nominal_value=1  v_nominal_unit=V
  diode : fl_lib/Electrical/Electrical Elements/Diode  Vf=Vdon_diode V  Ron=Rdon_diode Ohm  Goff=1e-8 1/Ohm  i_specify=off  i_priority=None  i=0 A  i_nominal_specify=off  i_nominal_value=1  i_nominal_unit=A  v_specify=off  v_priority=None  v=0 V  v_nominal_specify=off  v_nominal_value=1  v_nominal_unit=V
  RC snubber : fl_lib/Electrical/Electrical Elements/Capacitor  c=Csnubber F  r=Rsnubber Ohm  g=0 1/Ohm  i_specify=off  i_priority=None  i=0 A  i_nominal_specify=off  i_nominal_value=1  i_nominal_unit=A  v_specify=off  v_priority=None  v=0 V  v_nominal_specify=off  v_nominal_value=1  v_nominal_unit=V  vc_specify=off  vc_priority=High  vc=0 V  vc_nominal_specify=off  vc_nominal_value=1  vc_nominal_unit=V
  v_sensor : fl_lib/Electrical/Electrical Sensors/Voltage Sensor
  E : PMIOPort  Port=2  Side=Right
  i_A : nesl_utility/PS-Simulink Converter  PhysicalDomain=network_engine_domain  SubClassName=ps_output  LeftPortType=input  RightPortType=output  PseudoPeriodic=off  Frequencies=[]  VectorFormat=1-D array  Unit=A  AffineConversion=off
  v_V : nesl_utility/PS-Simulink Converter  PhysicalDomain=network_engine_domain  SubClassName=ps_output  LeftPortType=input  RightPortType=output  PseudoPeriodic=off  Frequencies=[]  VectorFormat=1-D array  Unit=V  AffineConversion=off
  i : Outport
  v : Outport  Port=2
  wires:
  g/1 -> gate/1
  i_A/1 -> i/1
  v_V/1 -> v/1
  connections:
  gate/RConn1 -- switch/RConn1
  C/RConn1 -- i_sensor/LConn1
  i_sensor/RConn2 -- switch/RConn2 -- diode/RConn1 -- RC snubber/LConn1 -- v_sensor/LConn1
  switch/LConn1 -- diode/LConn1 -- RC snubber/RConn1 -- v_sensor/RConn2 -- E/RConn1
  i_sensor/RConn1 -- i_A/LConn1
  v_sensor/RConn1 -- v_V/LConn1

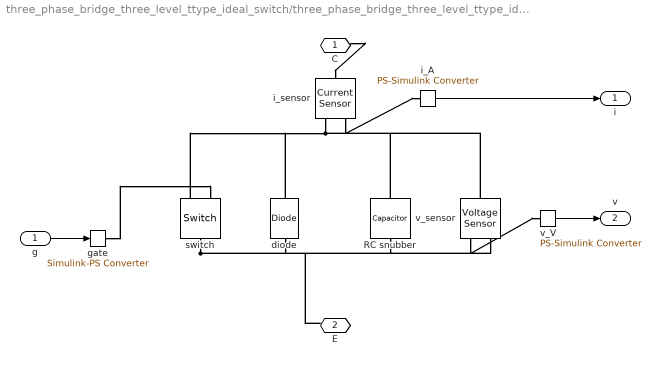
== system three_phase_bridge_three_level_ttype_ideal_switch/three_phase_bridge_three_level_ttype_ideal_switch/Q10 ==
  g : Inport
  gate : nesl_utility/Simulink-PS Converter  PhysicalDomain=network_engine_domain  SubClassName=ps_input  LeftPortType=input  RightPortType=output  PseudoPeriodic=off  Frequencies=[]  NoiseDistribution=none  NoiseParameters=[]  Unit=1  AffineConversion=off  FilteringAndDerivatives=provide  SimscapeFilterOrder=1  InputFilterTimeConstant=0.001  UdotUserProvided=0
  C : PMIOPort  Side=Left
  i_sensor : fl_lib/Electrical/Electrical Sensors/Current Sensor
  switch : fl_lib/Electrical/Electrical Elements/Switch  R_closed=Rds_on Ohm  G_open=1e-8 1/Ohm  Threshold=Vth  i_specify=off  i_priority=None  i=0 A  i_nominal_specify=off  i_nominal_value=1  i_nominal_unit=A  v_specify=off  v_priority=None  v=0 V  v_nominal_specify=off  v_nominal_value=1  v_nominal_unit=V
  diode : fl_lib/Electrical/Electrical Elements/Diode  Vf=Vdon_diode V  Ron=Rdon_diode Ohm  Goff=1e-8 1/Ohm  i_specify=off  i_priority=None  i=0 A  i_nominal_specify=off  i_nominal_value=1  i_nominal_unit=A  v_specify=off  v_priority=None  v=0 V  v_nominal_specify=off  v_nominal_value=1  v_nominal_unit=V
  RC snubber : fl_lib/Electrical/Electrical Elements/Capacitor  c=Csnubber F  r=Rsnubber Ohm  g=0 1/Ohm  i_specify=off  i_priority=None  i=0 A  i_nominal_specify=off  i_nominal_value=1  i_nominal_unit=A  v_specify=off  v_priority=None  v=0 V  v_nominal_specify=off  v_nominal_value=1  v_nominal_unit=V  vc_specify=off  vc_priority=High  vc=0 V  vc_nominal_specify=off  vc_nominal_value=1  vc_nominal_unit=V
  v_sensor : fl_lib/Electrical/Electrical Sensors/Voltage Sensor
  E : PMIOPort  Port=2  Side=Right
  i_A : nesl_utility/PS-Simulink Converter  PhysicalDomain=network_engine_domain  SubClassName=ps_output  LeftPortType=input  RightPortType=output  PseudoPeriodic=off  Frequencies=[]  VectorFormat=1-D array  Unit=A  AffineConversion=off
  v_V : nesl_utility/PS-Simulink Converter  PhysicalDomain=network_engine_domain  SubClassName=ps_output  LeftPortType=input  RightPortType=output  PseudoPeriodic=off  Frequencies=[]  VectorFormat=1-D array  Unit=V  AffineConversion=off
  i : Outport
  v : Outport  Port=2
  wires:
  g/1 -> gate/1
  i_A/1 -> i/1
  v_V/1 -> v/1
  connections:
  gate/RConn1 -- switch/RConn1
  C/RConn1 -- i_sensor/LConn1
  i_sensor/RConn2 -- switch/RConn2 -- diode/RConn1 -- RC snubber/LConn1 -- v_sensor/LConn1
  switch/LConn1 -- diode/LConn1 -- RC snubber/RConn1 -- v_sensor/RConn2 -- E/RConn1
  i_sensor/RConn1 -- i_A/LConn1
  v_sensor/RConn1 -- v_V/LConn1

== system three_phase_bridge_three_level_ttype_ideal_switch/three_phase_bridge_three_level_ttype_ideal_switch/Q11 ==
  g : Inport
  gate : nesl_utility/Simulink-PS Converter  PhysicalDomain=network_engine_domain  SubClassName=ps_input  LeftPortType=input  RightPortType=output  PseudoPeriodic=off  Frequencies=[]  NoiseDistribution=none  NoiseParameters=[]  Unit=1  AffineConversion=off  FilteringAndDerivatives=provide  SimscapeFilterOrder=1  InputFilterTimeConstant=0.001  UdotUserProvided=0
  C : PMIOPort  Side=Left
  i_sensor : fl_lib/Electrical/Electrical Sensors/Current Sensor
  switch : fl_lib/Electrical/Electrical Elements/Switch  R_closed=Rds_on Ohm  G_open=1e-8 1/Ohm  Threshold=Vth  i_specify=off  i_priority=None  i=0 A  i_nominal_specify=off  i_nominal_value=1  i_nominal_unit=A  v_specify=off  v_priority=None  v=0 V  v_nominal_specify=off  v_nominal_value=1  v_nominal_unit=V
  diode : fl_lib/Electrical/Electrical Elements/Diode  Vf=Vdon_diode V  Ron=Rdon_diode Ohm  Goff=1e-8 1/Ohm  i_specify=off  i_priority=None  i=0 A  i_nominal_specify=off  i_nominal_value=1  i_nominal_unit=A  v_specify=off  v_priority=None  v=0 V  v_nominal_specify=off  v_nominal_value=1  v_nominal_unit=V
  RC snubber : fl_lib/Electrical/Electrical Elements/Capacitor  c=Csnubber F  r=Rsnubber Ohm  g=0 1/Ohm  i_specify=off  i_priority=None  i=0 A  i_nominal_specify=off  i_nominal_value=1  i_nominal_unit=A  v_specify=off  v_priority=None  v=0 V  v_nominal_specify=off  v_nominal_value=1  v_nominal_unit=V  vc_specify=off  vc_priority=High  vc=0 V  vc_nominal_specify=off  vc_nominal_value=1  vc_nominal_unit=V
  v_sensor : fl_lib/Electrical/Electrical Sensors/Voltage Sensor
  E : PMIOPort  Port=2  Side=Right
  i_A : nesl_utility/PS-Simulink Converter  PhysicalDomain=network_engine_domain  SubClassName=ps_output  LeftPortType=input  RightPortType=output  PseudoPeriodic=off  Frequencies=[]  VectorFormat=1-D array  Unit=A  AffineConversion=off
  v_V : nesl_utility/PS-Simulink Converter  PhysicalDomain=network_engine_domain  SubClassName=ps_output  LeftPortType=input  RightPortType=output  PseudoPeriodic=off  Frequencies=[]  VectorFormat=1-D array  Unit=V  AffineConversion=off
  i : Outport
  v : Outport  Port=2
  wires:
  g/1 -> gate/1
  i_A/1 -> i/1
  v_V/1 -> v/1
  connections:
  gate/RConn1 -- switch/RConn1
  C/RConn1 -- i_sensor/LConn1
  i_sensor/RConn2 -- switch/RConn2 -- diode/RConn1 -- RC snubber/LConn1 -- v_sensor/LConn1
  switch/LConn1 -- diode/LConn1 -- RC snubber/RConn1 -- v_sensor/RConn2 -- E/RConn1
  i_sensor/RConn1 -- i_A/LConn1
  v_sensor/RConn1 -- v_V/LConn1

== system three_phase_bridge_three_level_ttype_ideal_switch/three_phase_bridge_three_level_ttype_ideal_switch/Q12 ==
  g : Inport
  gate : nesl_utility/Simulink-PS Converter  PhysicalDomain=network_engine_domain  SubClassName=ps_input  LeftPortType=input  RightPortType=output  PseudoPeriodic=off  Frequencies=[]  NoiseDistribution=none  NoiseParameters=[]  Unit=1  AffineConversion=off  FilteringAndDerivatives=provide  SimscapeFilterOrder=1  InputFilterTimeConstant=0.001  UdotUserProvided=0
  C : PMIOPort  Side=Left
  i_sensor : fl_lib/Electrical/Electrical Sensors/Current Sensor
  switch : fl_lib/Electrical/Electrical Elements/Switch  R_closed=Rds_on Ohm  G_open=1e-8 1/Ohm  Threshold=Vth  i_specify=off  i_priority=None  i=0 A  i_nominal_specify=off  i_nominal_value=1  i_nominal_unit=A  v_specify=off  v_priority=None  v=0 V  v_nominal_specify=off  v_nominal_value=1  v_nominal_unit=V
  diode : fl_lib/Electrical/Electrical Elements/Diode  Vf=Vdon_diode V  Ron=Rdon_diode Ohm  Goff=1e-8 1/Ohm  i_specify=off  i_priority=None  i=0 A  i_nominal_specify=off  i_nominal_value=1  i_nominal_unit=A  v_specify=off  v_priority=None  v=0 V  v_nominal_specify=off  v_nominal_value=1  v_nominal_unit=V
  RC snubber : fl_lib/Electrical/Electrical Elements/Capacitor  c=Csnubber F  r=Rsnubber Ohm  g=0 1/Ohm  i_specify=off  i_priority=None  i=0 A  i_nominal_specify=off  i_nominal_value=1  i_nominal_unit=A  v_specify=off  v_priority=None  v=0 V  v_nominal_specify=off  v_nominal_value=1  v_nominal_unit=V  vc_specify=off  vc_priority=High  vc=0 V  vc_nominal_specify=off  vc_nominal_value=1  vc_nominal_unit=V
  v_sensor : fl_lib/Electrical/Electrical Sensors/Voltage Sensor
  E : PMIOPort  Port=2  Side=Right
  i_A : nesl_utility/PS-Simulink Converter  PhysicalDomain=network_engine_domain  SubClassName=ps_output  LeftPortType=input  RightPortType=output  PseudoPeriodic=off  Frequencies=[]  VectorFormat=1-D array  Unit=A  AffineConversion=off
  v_V : nesl_utility/PS-Simulink Converter  PhysicalDomain=network_engine_domain  SubClassName=ps_output  LeftPortType=input  RightPortType=output  PseudoPeriodic=off  Frequencies=[]  VectorFormat=1-D array  Unit=V  AffineConversion=off
  i : Outport
  v : Outport  Port=2
  wires:
  g/1 -> gate/1
  i_A/1 -> i/1
  v_V/1 -> v/1
  connections:
  gate/RConn1 -- switch/RConn1
  C/RConn1 -- i_sensor/LConn1
  i_sensor/RConn2 -- switch/RConn2 -- diode/RConn1 -- RC snubber/LConn1 -- v_sensor/LConn1
  switch/LConn1 -- diode/LConn1 -- RC snubber/RConn1 -- v_sensor/RConn2 -- E/RConn1
  i_sensor/RConn1 -- i_A/LConn1
  v_sensor/RConn1 -- v_V/LConn1
